simulink model "Koudruped_simcape"  (R2025b)
settings: Solver=VariableStepAuto  StartTime=0.0  StopTime=30  RelTol=1e-2
undefined symbols (not defined in the file or in its folder): fractalcoef, smiData, X, Y, Z
libraries: sm_lib x589, nesl_utility x93, slpidlib x5, mspsensorlib x4, simulink_extras x4, mspfiltlib x3, simulink x2
(part 3 of 16)

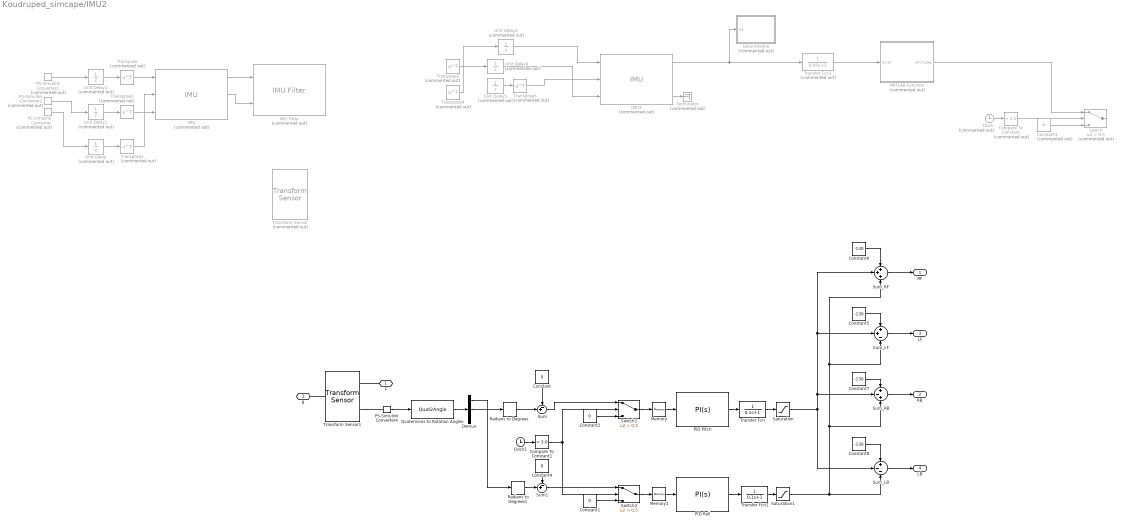
== system Koudruped_simcape/IMU2 ==
  Clock : Clock  Commented=on
  Clock1 : Clock
  Compare To Constant : simulink/Logic and Bit Operations/Compare To Constant  Commented=on  relop=>  const=3.0  OutDataTypeStr=boolean
  Compare To Constant1 : simulink/Logic and Bit Operations/Compare To Constant  relop=>  const=3.0  OutDataTypeStr=boolean
  Constant{,1..2,4} (4 alike) : Constant  Value=0
  Constant3 : Constant  Commented=on  Value=0
  Constant{5..8} (4 alike) : Constant  Value=-130
  Demux : Demux  Outputs=3
  Görüntüleme : Subsystem  Commented=on
  IMU : mspsensorlib/IMU  Commented=on  DispRefFrame=NED  TemperaturePort=off  Temperature=25  MagneticFieldPort=off  MagneticFieldNED=[ 27.5550, -2.4169, -16.0849 ]  MagneticFieldENU=[ -2.4169, 27.5550, 16.0849 ]  SeedDouble=67  SimulateUsing=Interpreted execution  AccelParamsMeasurementRange=156.96  AccelParamsResolution=0  AccelParamsConstantBias=[ 0.588, 0.588, 0.588 ]  AccelParamsAxesMisalignment=[ 100, 0, 0; 0, 100, 0; 0, 0, 100 ]  AccelParamsNoiseDensity=[ 0.00294, 0.00294, 0.00294 ]  AccelParamsBiasInstability=[ 0, 0, 0 ]  AccelParamsBiasInstabilityNumerator=fractalcoef().Numerator  AccelParamsBiasInstabilityDenominator=fractalcoef().Denominator  AccelParamsRandomWalk=[ 0, 0, 0 ]  AccelParamsNoiseType=double-sided  AccelParamsTemperatureBias=[ 0, 0, 0 ]  AccelParamsTemperatureScaleFactor=[ 0, 0, 0 ]  GyroParamsMeasurementRange=34.9  GyroParamsResolution=0  GyroParamsConstantBias=[ 0.0872, 0.0872, 0.0872 ]  GyroParamsAxesMisalignment=[ 100, 0, 0; 0, 100, 0; 0, 0, 100 ]  GyroParamsAccelerationBias=[ 0, 0, 0 ]  GyroParamsNoiseDensity=[ 0.0001745, 0.0001745, 0.0001745 ]  GyroParamsBiasInstability=[ 0, 0, 0 ]  GyroParamsBiasInstabilityNumerator=fractalcoef().Numerator  GyroParamsBiasInstabilityDenominator=fractalcoef().Denominator  GyroParamsRandomWalk=[ 0, 0, 0 ]  GyroParamsNoiseType=double-sided  GyroParamsTemperatureBias=[ 0, 0, 0 ]  GyroParamsTemperatureScaleFactor=[ 0, 0, 0 ]  MagParamsMeasurementRange=Inf  MagParamsResolution=0  MagParamsConstantBias=[ 0, 0, 0 ]  MagParamsAxesMisalignment=[ 100, 0, 0; 0, 100, 0; 0, 0, 100 ]  MagParamsNoiseDensity=[ 0, 0, 0 ]  MagParamsBiasInstability=[ 0, 0, 0 ]  MagParamsBiasInstabilityNumerator=fractalcoef().Numerator  MagParamsBiasInstabilityDenominator=fractalcoef().Denominator  MagParamsRandomWalk=[ 0, 0, 0 ]  MagParamsNoiseType=double-sided  MagParamsTemperatureBias=[ 0, 0, 0 ]  MagParamsTemperatureScaleFactor=[ 0, 0, 0 ]
  IMU Filter : mspfiltlib/IMU Filter  Commented=on  DispRefFrame=ENU  OrientationFormat=Rotation matrix  DecimationFactor=1  InitialProcessNoise=imufilter.defaultProcessNoise  AccelerometerNoise=8.64e-6  GyroscopeNoise=3.04e-8  GyroscopeDriftNoise=3.04e-13  LinearAccelerationNoise=0.0096236100000000012  LinearAccelerationDecayFactor=0.5  SimulateUsing=Interpreted execution
  IMU3 : mspsensorlib/IMU  Commented=on  DispRefFrame=ENU  TemperaturePort=off  Temperature=25  MagneticFieldPort=off  MagneticFieldNED=[ 27.5550, -2.4169, -16.0849 ]  MagneticFieldENU=[ -2.4169, 27.5550, 16.0849 ]  SeedDouble=67  SimulateUsing=Interpreted execution  AccelParamsMeasurementRange=19.6133  AccelParamsResolution=5.9855e-4  AccelParamsConstantBias=[ 0.19, 0.19, 0.19 ]  AccelParamsAxesMisalignment=[ 100, 0, 0; 0, 100, 0; 0, 0, 100 ]  AccelParamsNoiseDensity=[0.00294, 0.00294, 0.00294]  AccelParamsBiasInstability=[0.0004, 0.0004, 0.0004]  AccelParamsBiasInstabilityNumerator=fractalcoef().Numerator  AccelParamsBiasInstabilityDenominator=fractalcoef().Denominator  AccelParamsRandomWalk=[ 0, 0, 0 ]  AccelParamsNoiseType=double-sided  AccelParamsTemperatureBias=[ 0, 0, 0 ]  AccelParamsTemperatureScaleFactor=[ 0, 0, 0 ]  GyroParamsMeasurementRange=4.3633  GyroParamsResolution=0.00109  GyroParamsConstantBias=[0.0545, 0.0545, 0.0545]  GyroParamsAxesMisalignment=[ 100, 0, 0; 0, 100, 0; 0, 0, 100 ]  GyroParamsAccelerationBias=[ 0, 0, 0 ]  GyroParamsNoiseDensity=[4.36e-4, 4.36e-4, 4.36e-4]  GyroParamsBiasInstability=[2.4e-5, 2.4e-5, 2.4e-5]  GyroParamsBiasInstabilityNumerator=fractalcoef().Numerator  GyroParamsBiasInstabilityDenominator=fractalcoef().Denominator  GyroParamsRandomWalk=[ 0, 0, 0 ]  GyroParamsNoiseType=double-sided  GyroParamsTemperatureBias=[ 0, 0, 0 ]  GyroParamsTemperatureScaleFactor=[ 0, 0, 0 ]  MagParamsMeasurementRange=Inf  MagParamsResolution=0  MagParamsConstantBias=[ 0, 0, 0 ]  MagParamsAxesMisalignment=[ 100, 0, 0; 0, 100, 0; 0, 0, 100 ]  MagParamsNoiseDensity=[ 0, 0, 0 ]  MagParamsBiasInstability=[ 0, 0, 0 ]  MagParamsBiasInstabilityNumerator=fractalcoef().Numerator  MagParamsBiasInstabilityDenominator=fractalcoef().Denominator  MagParamsRandomWalk=[ 0, 0, 0 ]  MagParamsNoiseType=double-sided  MagParamsTemperatureBias=[ 0, 0, 0 ]  MagParamsTemperatureScaleFactor=[ 0, 0, 0 ]
  MATLAB Function : MATLAB Function  Commented=on  TreatAsAtomicUnit=on
  Memory : Memory
  Memory1 : Memory
  PID Pitch : slpidlib/PID Controller  Controller=PI  Form=Parallel  TimeDomain=Continuous-time  UseExternalTs=off  SampleTime=-1  IntegratorMethod=Forward Euler  FilterMethod=Forward Euler  ControllerParametersSource=internal  P=2  I=0.4  UseKiTs=off  D=0.05  UseExternalDerivativeSource=off  N=100  UseFilter=on  TunerSelectOption=Transfer Function Based (PID Tuner App)  InitialConditionSource=internal  InitialConditionForIntegrator=0  InitialConditionForFilter=0  DifferentiatorICPrevScaledInput=0  ExternalReset=none  TrackingMode=off  Kt=1  LimitOutput=on  SatLimitsSource=internal  UpperSaturationLimit=40  LowerSaturationLimit=-40  LinearizeAsGain=on  AntiWindupMode=back-calculation  Kb=1  LimitIntegrator=off  UpperIntegratorSaturationLimit=inf  LowerIntegratorSaturationLimit=-inf  POutMin=[]  POutMax=[]  IOutMin=[]  IOutMax=[]  DOutMin=[]  DOutMax=[]  NOutMin=[]  NOutMax=[]  SumOutMin=[]  SumOutMax=[]  SaturationOutMin=[]  SaturationOutMax=[]  PParamMin=[]  PParamMax=[]  IParamMin=[]  IParamMax=[]  DParamMin=[]  DParamMax=[]  NParamMin=[]  NParamMax=[]  KbParamMin=[]  KbParamMax=[]  KtParamMin=[]  KtParamMax=[]  KbOutMin=[]  KbOutMax=[]  KtOutMin=[]  KtOutMax=[]  IntegratorOutMin=[]  IntegratorOutMax=[]  FilterOutMin=[]  FilterOutMax=[]  SumI1OutMin=[]  SumI1OutMax=[]  SumI2OutMin=[]  SumI2OutMax=[]  SumI3OutMin=[]  SumI3OutMax=[]  SumI4OutMin=[]  SumI4OutMax=[]  SumDOutMin=[]  SumDOutMax=[]  DifferentiatorOutMin=[]  DifferentiatorOutMax=[]  FilterDiffOutCoefMin=[]  FilterDiffOutCoefMax=[]  ReciprocalOutMin=[]  ReciprocalOutMax=[]  SumDenOutMin=[]  SumDenOutMax=[]  SumNumOutMin=[]  SumNumOutMax=[]  DivideOutMin=[]  DivideOutMax=[]  UdiffTsProdOutMin=[]  UdiffTsProdOutMax=[]  NTsProdOutMin=[]  NTsProdOutMax=[]  UintegralTsProdOutMin=[]  UintegralTsProdOutMax=[]  UngainTsProdOutMin=[]  UngainTsProdOutMax=[]  ClampingZeroOutDataTypeStr=Inherit: Inherit via back propagation  ClampingZeroOutMin=[]  ClampingZeroOutMax=[]  FilterDenConstantOutDataTypeStr=Inherit: Inherit via back propagation  FilterDenConstantOutMin=[]  FilterDenConstantOutMax=[]  PCopyOutDataTypeStr=Inherit: Inherit via back propagation  PCopyOutMin=[]  PCopyOutMax=[]  NCopyOutDataTypeStr=Inherit: Inherit via back propagation  NCopyOutMin=[]  NCopyOutMax=[]  IntegratorContinuousStateAttributes=''  IntegratorStateMustResolveToSignalObject=off  IntegratorRTWStateStorageClass=Auto  FilterContinuousStateAttributes=''  FilterStateMustResolveToSignalObject=off  FilterRTWStateStorageClass=Auto  ParallelPVariant=InternalParameters  IdealPVariant=Disabled  IVariant=InternalParameters  DVariant=Disabled  IntegratorVariant=Continuous  SatVariant=Enabled  AWVariant=BackCalculation  PCopyVariant=Disabled  TRVariant=Disabled  FdbkBlocksVariant=Forward  IdealPFdbkVariant=Disabled  SatFdbkVariant=Disabled  DerivativeFilterVariant=Disabled  NVariant=Disabled  NCopyVariant=Disabled_SignalSpec  FilterICVariant=Disabled  IntegratorICVariant=InternalICs  ExternalResetVariant=Disabled  TRSumVariant=Passthrough  SumFdbkVariant=Disabled  SumVariant=Sum_PI  TsampFilterVariant=InternalTs  TsampNgainVariant=Passthrough  TsampIntegralVariant=Disabled_SignalSpec  ExternalSaturationOutDataTypeStr=Inherit: Same as second input  DerivativeSourceVariant=Disabled  PreIntVariant=InternalPreInt
  PID Roll : slpidlib/PID Controller  Controller=PI  Form=Parallel  TimeDomain=Continuous-time  UseExternalTs=off  SampleTime=-1  IntegratorMethod=Forward Euler  FilterMethod=Forward Euler  ControllerParametersSource=internal  P=2  I=0.4  UseKiTs=off  D=0.05  UseExternalDerivativeSource=off  N=100  UseFilter=on  TunerSelectOption=Transfer Function Based (PID Tuner App)  InitialConditionSource=internal  InitialConditionForIntegrator=0  InitialConditionForFilter=0  DifferentiatorICPrevScaledInput=0  ExternalReset=none  TrackingMode=off  Kt=1  LimitOutput=on  SatLimitsSource=internal  UpperSaturationLimit=40  LowerSaturationLimit=-40  LinearizeAsGain=on  AntiWindupMode=back-calculation  Kb=1  LimitIntegrator=off  UpperIntegratorSaturationLimit=inf  LowerIntegratorSaturationLimit=-inf  POutMin=[]  POutMax=[]  IOutMin=[]  IOutMax=[]  DOutMin=[]  DOutMax=[]  NOutMin=[]  NOutMax=[]  SumOutMin=[]  SumOutMax=[]  SaturationOutMin=[]  SaturationOutMax=[]  PParamMin=[]  PParamMax=[]  IParamMin=[]  IParamMax=[]  DParamMin=[]  DParamMax=[]  NParamMin=[]  NParamMax=[]  KbParamMin=[]  KbParamMax=[]  KtParamMin=[]  KtParamMax=[]  KbOutMin=[]  KbOutMax=[]  KtOutMin=[]  KtOutMax=[]  IntegratorOutMin=[]  IntegratorOutMax=[]  FilterOutMin=[]  FilterOutMax=[]  SumI1OutMin=[]  SumI1OutMax=[]  SumI2OutMin=[]  SumI2OutMax=[]  SumI3OutMin=[]  SumI3OutMax=[]  SumI4OutMin=[]  SumI4OutMax=[]  SumDOutMin=[]  SumDOutMax=[]  DifferentiatorOutMin=[]  DifferentiatorOutMax=[]  FilterDiffOutCoefMin=[]  FilterDiffOutCoefMax=[]  ReciprocalOutMin=[]  ReciprocalOutMax=[]  SumDenOutMin=[]  SumDenOutMax=[]  SumNumOutMin=[]  SumNumOutMax=[]  DivideOutMin=[]  DivideOutMax=[]  UdiffTsProdOutMin=[]  UdiffTsProdOutMax=[]  NTsProdOutMin=[]  NTsProdOutMax=[]  UintegralTsProdOutMin=[]  UintegralTsProdOutMax=[]  UngainTsProdOutMin=[]  UngainTsProdOutMax=[]  ClampingZeroOutDataTypeStr=Inherit: Inherit via back propagation  ClampingZeroOutMin=[]  ClampingZeroOutMax=[]  FilterDenConstantOutDataTypeStr=Inherit: Inherit via back propagation  FilterDenConstantOutMin=[]  FilterDenConstantOutMax=[]  PCopyOutDataTypeStr=Inherit: Inherit via back propagation  PCopyOutMin=[]  PCopyOutMax=[]  NCopyOutDataTypeStr=Inherit: Inherit via back propagation  NCopyOutMin=[]  NCopyOutMax=[]  IntegratorContinuousStateAttributes=''  IntegratorStateMustResolveToSignalObject=off  IntegratorRTWStateStorageClass=Auto  FilterContinuousStateAttributes=''  FilterStateMustResolveToSignalObject=off  FilterRTWStateStorageClass=Auto  ParallelPVariant=InternalParameters  IdealPVariant=Disabled  IVariant=InternalParameters  DVariant=Disabled  IntegratorVariant=Continuous  SatVariant=Enabled  AWVariant=BackCalculation  PCopyVariant=Disabled  TRVariant=Disabled  FdbkBlocksVariant=Forward  IdealPFdbkVariant=Disabled  SatFdbkVariant=Disabled  DerivativeFilterVariant=Disabled  NVariant=Disabled  NCopyVariant=Disabled_SignalSpec  FilterICVariant=Disabled  IntegratorICVariant=InternalICs  ExternalResetVariant=Disabled  TRSumVariant=Passthrough  SumFdbkVariant=Disabled  SumVariant=Sum_PI  TsampFilterVariant=InternalTs  TsampNgainVariant=Passthrough  TsampIntegralVariant=Disabled_SignalSpec  ExternalSaturationOutDataTypeStr=Inherit: Same as second input  DerivativeSourceVariant=Disabled  PreIntVariant=InternalPreInt
  PS-Simulink Converter : nesl_utility/PS-Simulink Converter  Commented=on  PhysicalDomain=network_engine_domain  SubClassName=ps_output  LeftPortType=input  RightPortType=output  PseudoPeriodic=off  Frequencies=[]  VectorFormat=inherit  Unit=inherit  AffineConversion=off
  PS-Simulink Converter1 : nesl_utility/PS-Simulink Converter  Commented=on  PhysicalDomain=network_engine_domain  SubClassName=ps_output  LeftPortType=input  RightPortType=output  PseudoPeriodic=off  Frequencies=[]  VectorFormat=inherit  Unit=inherit  AffineConversion=off
  PS-Simulink Converter2 : nesl_utility/PS-Simulink Converter  Commented=on  PhysicalDomain=network_engine_domain  SubClassName=ps_output  LeftPortType=input  RightPortType=output  PseudoPeriodic=off  Frequencies=[]  VectorFormat=inherit  Unit=inherit  AffineConversion=off
  PS-Simulink Converter4 : nesl_utility/PS-Simulink Converter  PhysicalDomain=network_engine_domain  SubClassName=ps_output  LeftPortType=input  RightPortType=output  PseudoPeriodic=off  Frequencies=[]  VectorFormat=inherit  Unit=inherit  AffineConversion=off
  Quaternions to Rotation Angles : Quat2Angle
      settings: AttributesFormatString=Rotation Order: %<rotationOrder>
  Radians to Degrees : simulink_extras/Transformations/Radians to Degrees
  Radians to Degrees1 : simulink_extras/Transformations/Radians to Degrees
  Saturation : Saturate  UpperLimit=+40  LowerLimit=-40
  Saturation1 : Saturate  UpperLimit=+40  LowerLimit=-40
  Sum : Sum  Inputs=-+|
  Sum1 : Sum  Inputs=-+|
  Sum_LB : Sum  Inputs=+--
  Sum_LF : Sum  Inputs=++-
  Sum_RB : Sum  Inputs=+-+
  Sum_RF : Sum  Inputs=+++
  Switch : Switch  Commented=on  Criteria=u2 > Threshold  Threshold=0.5  SaturateOnIntegerOverflow=off  InputSameDT=off
  Switch1 : Switch  Criteria=u2 > Threshold  Threshold=0.5  SaturateOnIntegerOverflow=off  InputSameDT=off
  Switch2 : Switch  Criteria=u2 > Threshold  Threshold=0.5  SaturateOnIntegerOverflow=off  InputSameDT=off
  Terminator : Terminator  Commented=on
  Transfer Fcn : TransferFcn  Denominator=[0.1 1]
  Transfer Fcn1 : TransferFcn  Commented=on  Denominator=[0.05 1]
  Transfer Fcn2 : TransferFcn  Denominator=[0.1 1]
  Transform Sensor : sm_lib/Frames and Transforms/Transform Sensor  Commented=on  MeasurementFrame=World  RotationSequence=ZYX  SenseAngle=off  SenseAxis=off  SenseQ=on  SenseR=off  SenseRotationSequence=off  SenseOmegaX=off  SenseOmegaY=off  SenseOmegaZ=off  SenseOmega=on  SenseQDot=off  SenseRDot=off  SenseRotationSequenceDot=off  SenseAlphaX=off  SenseAlphaY=off  SenseAlphaZ=off  SenseAlpha=off  SenseQDDot=off  SenseRDDot=off  SenseX=off  SenseY=off  SenseZ=off  SenseXYZ=off  SenseRad=off  SenseAzim=off  SenseDist=off  SenseInc=off  SenseXDot=off  SenseYDot=off  SenseZDot=off  SenseXYZDot=off  SenseRadDot=off  SenseAzimDot=off  SenseDistDot=off  SenseIncDot=off  SenseXDDot=off  SenseYDDot=off  SenseZDDot=off  SenseXYZDDot=on  SenseRadDDot=off  SenseAzimDDot=off  SenseDistDDot=off  SenseIncDDot=off
  Transform Sensor1 : sm_lib/Frames and Transforms/Transform Sensor  MeasurementFrame=World  RotationSequence=ZYX  SenseAngle=off  SenseAxis=off  SenseQ=on  SenseR=off  SenseRotationSequence=off  SenseOmegaX=off  SenseOmegaY=off  SenseOmegaZ=off  SenseOmega=off  SenseQDot=off  SenseRDot=off  SenseRotationSequenceDot=off  SenseAlphaX=off  SenseAlphaY=off  SenseAlphaZ=off  SenseAlpha=off  SenseQDDot=off  SenseRDDot=off  SenseX=off  SenseY=off  SenseZ=off  SenseXYZ=off  SenseRad=off  SenseAzim=off  SenseDist=off  SenseInc=off  SenseXDot=off  SenseYDot=off  SenseZDot=off  SenseXYZDot=off  SenseRadDot=off  SenseAzimDot=off  SenseDistDot=off  SenseIncDot=off  SenseXDDot=off  SenseYDDot=off  SenseZDDot=off  SenseXYZDDot=off  SenseRadDDot=off  SenseAzimDDot=off  SenseDistDDot=off  SenseIncDDot=off
  Transpose{,1..5} (6 alike) : Math  Commented=on  Operator=transpose
  Unit Delay : UnitDelay  Commented=on  SampleTime=-1  HasFrameUpgradeWarning=on
  Unit Delay1 : UnitDelay  Commented=on  InitialCondition="[1 0 0 ;0 0 0  ; 0 0 0 ]"  SampleTime=-1  HasFrameUpgradeWarning=on
  Unit Delay2 : UnitDelay  Commented=on  InitialCondition=[0 ;0 ;-9.81 ]  SampleTime=-1  HasFrameUpgradeWarning=on
  Unit Delay3 : UnitDelay  Commented=on  SampleTime=0.001  HasFrameUpgradeWarning=on
  Unit Delay4 : UnitDelay  Commented=on  SampleTime=0.001  HasFrameUpgradeWarning=on
  Unit Delay5 : UnitDelay  Commented=on  SampleTime=0.001  HasFrameUpgradeWarning=on
  F : PMIOPort  Side=Left
  B : PMIOPort  Port=2  Side=Left
  RF : Outport
  RB : Outport  Port=2
  LF : Outport  Port=3
  LB : Outport  Port=4
  wires:
  Constant/1 -> Sum/1
  PID Pitch/1 -> Transfer Fcn/1
  Demux/2 -> Radians to Degrees/1
  Quaternions to Rotation Angles/1 -> Demux/1
  Transpose2/1 -> IMU/3
  Unit Delay2/1 -> Transpose/1
  PS-Simulink Converter1/1 -> Unit Delay2/1
  PS-Simulink Converter2/1 -> Unit Delay1/1
  Unit Delay1/1 -> Transpose2/1
  PS-Simulink Converter/1 -> Unit Delay/1
  IMU/2 -> IMU Filter/2
  Unit Delay/1 -> Transpose1/1
  IMU/1 -> IMU Filter/1
  Transpose/1 -> IMU/1
  Transpose1/1 -> IMU/2
  Memory/1 -> PID Pitch/1
  Transfer Fcn/1 -> Saturation/1
  Transpose4/1 -> Unit Delay3/1
  Transpose3/1 -> IMU3/2
  Transpose5/1 -> Unit Delay4/1
  Unit Delay3/1 -> IMU3/1
  Unit Delay4/1 -> IMU3/3
  Unit Delay5/1 -> Transpose3/1
  IMU3/1 -> Transfer Fcn1/1, Görüntüleme/1(In1)
  IMU3/3 -> Terminator/1
  Compare To Constant/1 -> Switch/2
  Constant3/1 -> Switch/3
  Clock/1 -> Compare To Constant/1
  Transfer Fcn1/1 -> MATLAB Function/1(accel)
  MATLAB Function/1(pitch_deg) -> Switch/1
  Radians to Degrees/1 -> Sum/2
  PS-Simulink Converter4/1 -> Quaternions to Rotation Angles/1
  Radians to Degrees1/1 -> Sum1/2
  PID Roll/1 -> Transfer Fcn2/1
  Memory1/1 -> PID Roll/1
  Constant4/1 -> Sum1/1
  Transfer Fcn2/1 -> Saturation1/1
  Sum_RF/1 -> RF/1
  Sum_LF/1 -> LF/1
  Sum_RB/1 -> RB/1
  Sum_LB/1 -> LB/1
  Constant5/1 -> Sum_LF/1
  Constant6/1 -> Sum_RF/1
  Constant7/1 -> Sum_RB/1
  Constant8/1 -> Sum_LB/1
  Saturation/1 -> Sum_LB/2, Sum_LF/2, Sum_RF/2, Sum_RB/2
  Saturation1/1 -> Sum_RB/3, Sum_LF/3, Sum_RF/3, Sum_LB/3
  Clock1/1 -> Compare To Constant1/1
  Constant2/1 -> Switch1/3
  Switch2/1 -> Memory1/1
  Constant1/1 -> Switch2/3
  Compare To Constant1/1 -> Switch1/2, Switch2/2
  Switch1/1 -> Memory/1
  Sum/1 -> Switch1/1
  Sum1/1 -> Switch2/1
  Demux/1 -> Radians to Degrees1/1
  connections:
  Transform Sensor1/LConn1 -- B/RConn1
  Transform Sensor1/RConn2 -- PS-Simulink Converter4/LConn1
  F/RConn1 -- Transform Sensor1/RConn1

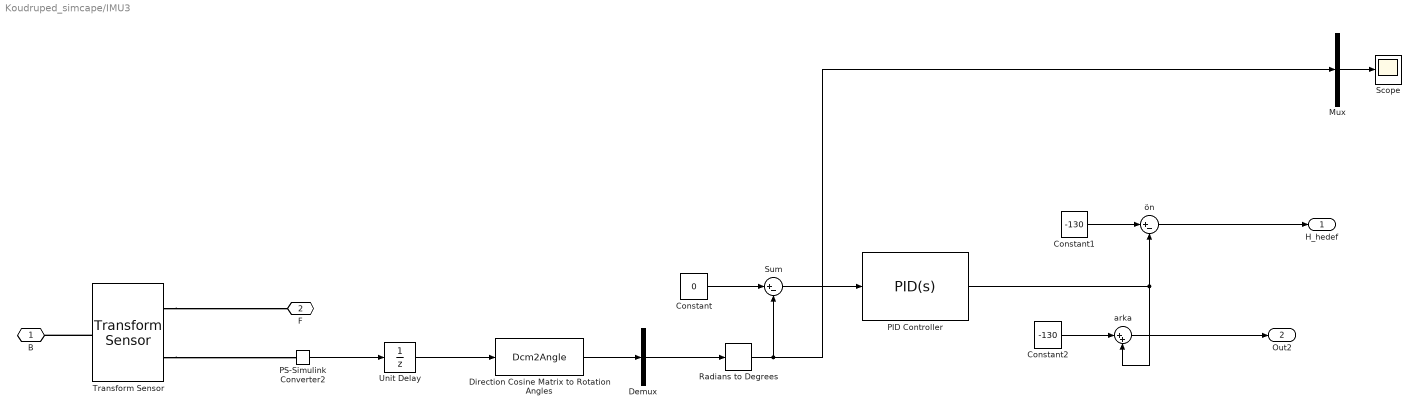
== system Koudruped_simcape/IMU3 ==
  Constant : Constant  Value=0
  Constant1 : Constant  Value=-130
  Constant2 : Constant  Value=-130
  Demux : Demux  Outputs=3
  Direction Cosine Matrix to Rotation Angles : Dcm2Angle
      settings: AttributesFormatString=Rotation Order: %<rotationOrder>
  Mux : Mux  Inputs=3
  PID Controller : slpidlib/PID Controller  Controller=PID  Form=Parallel  TimeDomain=Continuous-time  UseExternalTs=off  SampleTime=-1  IntegratorMethod=Forward Euler  FilterMethod=Forward Euler  ControllerParametersSource=internal  P=1  I=0.05  UseKiTs=off  D=0  UseExternalDerivativeSource=off  N=100  UseFilter=on  TunerSelectOption=Transfer Function Based (PID Tuner App)  InitialConditionSource=internal  InitialConditionForIntegrator=0  InitialConditionForFilter=0  DifferentiatorICPrevScaledInput=0  ExternalReset=none  TrackingMode=off  Kt=1  LimitOutput=off  SatLimitsSource=internal  UpperSaturationLimit=inf  LowerSaturationLimit=-inf  LinearizeAsGain=on  AntiWindupMode=none  Kb=1  LimitIntegrator=off  UpperIntegratorSaturationLimit=inf  LowerIntegratorSaturationLimit=-inf  POutMin=[]  POutMax=[]  IOutMin=[]  IOutMax=[]  DOutMin=[]  DOutMax=[]  NOutMin=[]  NOutMax=[]  SumOutMin=[]  SumOutMax=[]  SaturationOutMin=[]  SaturationOutMax=[]  PParamMin=[]  PParamMax=[]  IParamMin=[]  IParamMax=[]  DParamMin=[]  DParamMax=[]  NParamMin=[]  NParamMax=[]  KbParamMin=[]  KbParamMax=[]  KtParamMin=[]  KtParamMax=[]  KbOutMin=[]  KbOutMax=[]  KtOutMin=[]  KtOutMax=[]  IntegratorOutMin=[]  IntegratorOutMax=[]  FilterOutMin=[]  FilterOutMax=[]  SumI1OutMin=[]  SumI1OutMax=[]  SumI2OutMin=[]  SumI2OutMax=[]  SumI3OutMin=[]  SumI3OutMax=[]  SumI4OutMin=[]  SumI4OutMax=[]  SumDOutMin=[]  SumDOutMax=[]  DifferentiatorOutMin=[]  DifferentiatorOutMax=[]  FilterDiffOutCoefMin=[]  FilterDiffOutCoefMax=[]  ReciprocalOutMin=[]  ReciprocalOutMax=[]  SumDenOutMin=[]  SumDenOutMax=[]  SumNumOutMin=[]  SumNumOutMax=[]  DivideOutMin=[]  DivideOutMax=[]  UdiffTsProdOutMin=[]  UdiffTsProdOutMax=[]  NTsProdOutMin=[]  NTsProdOutMax=[]  UintegralTsProdOutMin=[]  UintegralTsProdOutMax=[]  UngainTsProdOutMin=[]  UngainTsProdOutMax=[]  ClampingZeroOutDataTypeStr=Inherit: Inherit via back propagation  ClampingZeroOutMin=[]  ClampingZeroOutMax=[]  FilterDenConstantOutDataTypeStr=Inherit: Inherit via back propagation  FilterDenConstantOutMin=[]  FilterDenConstantOutMax=[]  PCopyOutDataTypeStr=Inherit: Inherit via back propagation  PCopyOutMin=[]  PCopyOutMax=[]  NCopyOutDataTypeStr=Inherit: Inherit via back propagation  NCopyOutMin=[]  NCopyOutMax=[]  IntegratorContinuousStateAttributes=''  IntegratorStateMustResolveToSignalObject=off  IntegratorRTWStateStorageClass=Auto  FilterContinuousStateAttributes=''  FilterStateMustResolveToSignalObject=off  FilterRTWStateStorageClass=Auto  ParallelPVariant=InternalParameters  IdealPVariant=Disabled  IVariant=InternalParameters  DVariant=InternalParameters  IntegratorVariant=Continuous  SatVariant=Disabled  AWVariant=Passthrough  PCopyVariant=Disabled  TRVariant=Disabled  FdbkBlocksVariant=Forward  IdealPFdbkVariant=Disabled  SatFdbkVariant=Disabled  DerivativeFilterVariant=ContFilter  NVariant=InternalParameters  NCopyVariant=Disabled  FilterICVariant=InternalICsFilter  IntegratorICVariant=InternalICs  ExternalResetVariant=Disabled  TRSumVariant=Passthrough  SumFdbkVariant=Disabled  SumVariant=Sum_PID  TsampFilterVariant=InternalTs  TsampNgainVariant=Passthrough  TsampIntegralVariant=Disabled_SignalSpec  ExternalSaturationOutDataTypeStr=Inherit: Same as second input  DerivativeSourceVariant=ErrorSignal  PreIntVariant=InternalPreInt
  PS-Simulink Converter2 : nesl_utility/PS-Simulink Converter  PhysicalDomain=network_engine_domain  SubClassName=ps_output  LeftPortType=input  RightPortType=output  PseudoPeriodic=off  Frequencies=[]  VectorFormat=inherit  Unit=inherit  AffineConversion=off
  Radians to Degrees : simulink_extras/Transformations/Radians to Degrees
  Scope : Scope
      settings: ActiveDisplayYMinimum=-51.725776270156686  ActiveDisplayYMaximum=42.428044280294451  DataLoggingVariableName=ScopeData2
  Sum : Sum  Inputs=|+-
  Transform Sensor : sm_lib/Frames and Transforms/Transform Sensor  MeasurementFrame=World  RotationSequence=XYX  SenseAngle=off  SenseAxis=off  SenseQ=off  SenseR=on  SenseRotationSequence=off  SenseOmegaX=off  SenseOmegaY=off  SenseOmegaZ=off  SenseOmega=off  SenseQDot=off  SenseRDot=off  SenseRotationSequenceDot=off  SenseAlphaX=off  SenseAlphaY=off  SenseAlphaZ=off  SenseAlpha=off  SenseQDDot=off  SenseRDDot=off  SenseX=off  SenseY=off  SenseZ=off  SenseXYZ=off  SenseRad=off  SenseAzim=off  SenseDist=off  SenseInc=off  SenseXDot=off  SenseYDot=off  SenseZDot=off  SenseXYZDot=off  SenseRadDot=off  SenseAzimDot=off  SenseDistDot=off  SenseIncDot=off  SenseXDDot=off  SenseYDDot=off  SenseZDDot=off  SenseXYZDDot=off  SenseRadDDot=off  SenseAzimDDot=off  SenseDistDDot=off  SenseIncDDot=off
  Unit Delay : UnitDelay  SampleTime=-1  HasFrameUpgradeWarning=on
  arka : Sum  Inputs=|++
  ön : Sum  Inputs=|+-
  B : PMIOPort  Side=Left
  F : PMIOPort  Port=2  Side=Left
  H_hedef : Outport
  Out2 : Outport  Port=2
  wires:
  ön/1 -> H_hedef/1
  Constant/1 -> Sum/1
  Constant2/1 -> arka/1
  Constant1/1 -> ön/1
  PID Controller/1 -> ön/2, arka/2
  Sum/1 -> PID Controller/1
  Demux/2 -> Radians to Degrees/1
  Direction Cosine Matrix to Rotation Angles/1 -> Demux/1
  Radians to Degrees/1 -> Mux/2, Sum/2
  PS-Simulink Converter2/1 -> Unit Delay/1
  Unit Delay/1 -> Direction Cosine Matrix to Rotation Angles/1
  arka/1 -> Out2/1
  Mux/1 -> Scope/1
  connections:
  Transform Sensor/RConn2 -- PS-Simulink Converter2/LConn1
  Transform Sensor/LConn1 -- B/RConn1
  Transform Sensor/RConn1 -- F/RConn1

== system Koudruped_simcape/Left Back Step ==
  H_hedef : Inport
  Clock1 : Clock
  Constant : Constant  Value=0
  Demux1 : Demux  Outputs=3
  Gain : Gain  Gain=-1
  MATLAB Function1 : MATLAB Function  TreatAsAtomicUnit=on
  MATLAB Function2 : MATLAB Function  TreatAsAtomicUnit=on
  Simulink-PS Converter1 : nesl_utility/Simulink-PS Converter  PhysicalDomain=network_engine_domain  SubClassName=ps_input  LeftPortType=input  RightPortType=output  PseudoPeriodic=off  Frequencies=[]  NoiseDistribution=none  NoiseParameters=[]  Unit=deg  AffineConversion=off  FilteringAndDerivatives=filter  SimscapeFilterOrder=2  InputFilterTimeConstant=0.001  UdotUserProvided=0
  Simulink-PS Converter2 : nesl_utility/Simulink-PS Converter  PhysicalDomain=network_engine_domain  SubClassName=ps_input  LeftPortType=input  RightPortType=output  PseudoPeriodic=off  Frequencies=[]  NoiseDistribution=none  NoiseParameters=[]  Unit=deg  AffineConversion=off  FilteringAndDerivatives=filter  SimscapeFilterOrder=2  InputFilterTimeConstant=0.001  UdotUserProvided=0
  Simulink-PS Converter3 : nesl_utility/Simulink-PS Converter  PhysicalDomain=network_engine_domain  SubClassName=ps_input  LeftPortType=input  RightPortType=output  PseudoPeriodic=off  Frequencies=[]  NoiseDistribution=none  NoiseParameters=[]  Unit=deg  AffineConversion=off  FilteringAndDerivatives=filter  SimscapeFilterOrder=2  InputFilterTimeConstant=0.001  UdotUserProvided=0
  Mafsal 1 : PMIOPort  Side=Right
  Mafsal 2 : PMIOPort  Port=2  Side=Right
  Mafsal 3 : PMIOPort  Port=3  Side=Right
  wires:
  Clock1/1 -> MATLAB Function1/1(t)
  Constant/1 -> MATLAB Function1/2(phase_offset)
  MATLAB Function1/1(pos) -> MATLAB Function2/1(pos)
  Demux1/2 -> Simulink-PS Converter1/1
  Demux1/3 -> Simulink-PS Converter2/1
  Demux1/1 -> Gain/1
  MATLAB Function2/1(angles) -> Demux1/1
  H_hedef/1 -> MATLAB Function1/3(H_hedef)
  Gain/1 -> Simulink-PS Converter3/1
  connections:
  Mafsal 1/RConn1 -- Simulink-PS Converter3/RConn1
  Simulink-PS Converter1/RConn1 -- Mafsal 2/RConn1
  Simulink-PS Converter2/RConn1 -- Mafsal 3/RConn1

== system Koudruped_simcape/Left Back Step1 ==
  H_hedef : Inport
  Clock1 : Clock
  Constant : Constant  Value=0
  Demux1 : Demux  Outputs=3
  Gain : Gain  Gain=-1
  MATLAB Function1 : MATLAB Function  TreatAsAtomicUnit=on
  MATLAB Function2 : MATLAB Function  TreatAsAtomicUnit=on
  Simulink-PS Converter1 : nesl_utility/Simulink-PS Converter  PhysicalDomain=network_engine_domain  SubClassName=ps_input  LeftPortType=input  RightPortType=output  PseudoPeriodic=off  Frequencies=[]  NoiseDistribution=none  NoiseParameters=[]  Unit=deg  AffineConversion=off  FilteringAndDerivatives=filter  SimscapeFilterOrder=2  InputFilterTimeConstant=0.001  UdotUserProvided=0
  Simulink-PS Converter2 : nesl_utility/Simulink-PS Converter  PhysicalDomain=network_engine_domain  SubClassName=ps_input  LeftPortType=input  RightPortType=output  PseudoPeriodic=off  Frequencies=[]  NoiseDistribution=none  NoiseParameters=[]  Unit=deg  AffineConversion=off  FilteringAndDerivatives=filter  SimscapeFilterOrder=2  InputFilterTimeConstant=0.001  UdotUserProvided=0
  Simulink-PS Converter3 : nesl_utility/Simulink-PS Converter  PhysicalDomain=network_engine_domain  SubClassName=ps_input  LeftPortType=input  RightPortType=output  PseudoPeriodic=off  Frequencies=[]  NoiseDistribution=none  NoiseParameters=[]  Unit=deg  AffineConversion=off  FilteringAndDerivatives=filter  SimscapeFilterOrder=2  InputFilterTimeConstant=0.001  UdotUserProvided=0
  Mafsal 1 : PMIOPort  Side=Right
  Mafsal 2 : PMIOPort  Port=2  Side=Right
  Mafsal 3 : PMIOPort  Port=3  Side=Right
  wires:
  Clock1/1 -> MATLAB Function1/1(t)
  Constant/1 -> MATLAB Function1/2(phase_offset)
  MATLAB Function1/1(pos) -> MATLAB Function2/1(pos)
  Demux1/2 -> Simulink-PS Converter1/1
  Demux1/1 -> Gain/1
  MATLAB Function2/1(angles) -> Demux1/1
  H_hedef/1 -> MATLAB Function1/3(H_hedef)
  Gain/1 -> Simulink-PS Converter3/1
  Demux1/3 -> Simulink-PS Converter2/1
  connections:
  Mafsal 1/RConn1 -- Simulink-PS Converter3/RConn1
  Simulink-PS Converter1/RConn1 -- Mafsal 2/RConn1
  Simulink-PS Converter2/RConn1 -- Mafsal 3/RConn1

== system Koudruped_simcape/Left Back Step2 ==
  H_hedef : Inport
  Clock1 : Clock
  Constant : Constant  Value=0
  Demux1 : Demux  Outputs=3
  Display : Display
  Gain : Gain  Gain=-1
  Left Back : Scope
      settings: ActiveDisplayYMinimum=-1  ActiveDisplayYMaximum=1  DataLoggingVariableName=ScopeData4
  Left Back1 : Scope
      settings: ActiveDisplayYMinimum=-1  ActiveDisplayYMaximum=1  DataLoggingVariableName=ScopeData5
  MATLAB Function1 : MATLAB Function  TreatAsAtomicUnit=on
  MATLAB Function2 : MATLAB Function  TreatAsAtomicUnit=on
  Simulink-PS Converter1 : nesl_utility/Simulink-PS Converter  PhysicalDomain=network_engine_domain  SubClassName=ps_input  LeftPortType=input  RightPortType=output  PseudoPeriodic=off  Frequencies=[]  NoiseDistribution=none  NoiseParameters=[]  Unit=deg  AffineConversion=off  FilteringAndDerivatives=filter  SimscapeFilterOrder=2  InputFilterTimeConstant=0.001  UdotUserProvided=0
  Simulink-PS Converter2 : nesl_utility/Simulink-PS Converter  PhysicalDomain=network_engine_domain  SubClassName=ps_input  LeftPortType=input  RightPortType=output  PseudoPeriodic=off  Frequencies=[]  NoiseDistribution=none  NoiseParameters=[]  Unit=deg  AffineConversion=off  FilteringAndDerivatives=filter  SimscapeFilterOrder=2  InputFilterTimeConstant=0.001  UdotUserProvided=0
  Simulink-PS Converter3 : nesl_utility/Simulink-PS Converter  PhysicalDomain=network_engine_domain  SubClassName=ps_input  LeftPortType=input  RightPortType=output  PseudoPeriodic=off  Frequencies=[]  NoiseDistribution=none  NoiseParameters=[]  Unit=deg  AffineConversion=off  FilteringAndDerivatives=filter  SimscapeFilterOrder=2  InputFilterTimeConstant=0.001  UdotUserProvided=0
  Mafsal 1 : PMIOPort  Side=Right
  Mafsal 2 : PMIOPort  Port=2  Side=Right
  Mafsal 3 : PMIOPort  Port=3  Side=Right
  wires:
  Clock1/1 -> MATLAB Function1/1(t)
  Constant/1 -> MATLAB Function1/2(phase_offset)
  MATLAB Function1/1(pos) -> MATLAB Function2/1(pos)
  Demux1/2 -> Simulink-PS Converter1/1
  Demux1/1 -> Gain/1
  MATLAB Function2/1(angles) -> Demux1/1
  H_hedef/1 -> Display/1, Left Back/1, MATLAB Function1/3(H_hedef)
  Gain/1 -> Simulink-PS Converter3/1
  Demux1/3 -> Left Back1/1, Simulink-PS Converter2/1
  connections:
  Mafsal 1/RConn1 -- Simulink-PS Converter3/RConn1
  Simulink-PS Converter1/RConn1 -- Mafsal 2/RConn1
  Simulink-PS Converter2/RConn1 -- Mafsal 3/RConn1

== system Koudruped_simcape/Left Back Step3 ==
  H_hedef : Inport
  Clock1 : Clock
  Constant : Constant  Value=0
  Demux1 : Demux  Outputs=3
  Gain : Gain  Gain=-1
  MATLAB Function1 : MATLAB Function  TreatAsAtomicUnit=on
  MATLAB Function2 : MATLAB Function  TreatAsAtomicUnit=on
  Simulink-PS Converter1 : nesl_utility/Simulink-PS Converter  PhysicalDomain=network_engine_domain  SubClassName=ps_input  LeftPortType=input  RightPortType=output  PseudoPeriodic=off  Frequencies=[]  NoiseDistribution=none  NoiseParameters=[]  Unit=deg  AffineConversion=off  FilteringAndDerivatives=filter  SimscapeFilterOrder=2  InputFilterTimeConstant=0.001  UdotUserProvided=0
  Simulink-PS Converter2 : nesl_utility/Simulink-PS Converter  PhysicalDomain=network_engine_domain  SubClassName=ps_input  LeftPortType=input  RightPortType=output  PseudoPeriodic=off  Frequencies=[]  NoiseDistribution=none  NoiseParameters=[]  Unit=deg  AffineConversion=off  FilteringAndDerivatives=filter  SimscapeFilterOrder=2  InputFilterTimeConstant=0.001  UdotUserProvided=0
  Simulink-PS Converter3 : nesl_utility/Simulink-PS Converter  PhysicalDomain=network_engine_domain  SubClassName=ps_input  LeftPortType=input  RightPortType=output  PseudoPeriodic=off  Frequencies=[]  NoiseDistribution=none  NoiseParameters=[]  Unit=deg  AffineConversion=off  FilteringAndDerivatives=filter  SimscapeFilterOrder=2  InputFilterTimeConstant=0.001  UdotUserProvided=0
  Mafsal 1 : PMIOPort  Side=Right
  Mafsal 2 : PMIOPort  Port=2  Side=Right
  Mafsal 3 : PMIOPort  Port=3  Side=Right
  wires:
  Clock1/1 -> MATLAB Function1/1(t)
  Constant/1 -> MATLAB Function1/2(phase_offset)
  MATLAB Function1/1(pos) -> MATLAB Function2/1(pos)
  Demux1/2 -> Simulink-PS Converter1/1
  Demux1/1 -> Gain/1
  MATLAB Function2/1(angles) -> Demux1/1
  H_hedef/1 -> MATLAB Function1/3(H_hedef)
  Gain/1 -> Simulink-PS Converter3/1
  Demux1/3 -> Simulink-PS Converter2/1
  connections:
  Mafsal 1/RConn1 -- Simulink-PS Converter3/RConn1
  Simulink-PS Converter1/RConn1 -- Mafsal 2/RConn1
  Simulink-PS Converter2/RConn1 -- Mafsal 3/RConn1

== system Koudruped_simcape/Left Front Step ==
  H_hedef : Inport
  Clock1 : Clock
  Constant : Constant  Value=0.5
  Demux1 : Demux  Outputs=3
  Gain : Gain  Gain=-1
  MATLAB Function1 : MATLAB Function  TreatAsAtomicUnit=on
  MATLAB Function2 : MATLAB Function  TreatAsAtomicUnit=on
  Simulink-PS Converter1 : nesl_utility/Simulink-PS Converter  PhysicalDomain=network_engine_domain  SubClassName=ps_input  LeftPortType=input  RightPortType=output  PseudoPeriodic=off  Frequencies=[]  NoiseDistribution=none  NoiseParameters=[]  Unit=deg  AffineConversion=off  FilteringAndDerivatives=filter  SimscapeFilterOrder=2  InputFilterTimeConstant=0.001  UdotUserProvided=0
  Simulink-PS Converter2 : nesl_utility/Simulink-PS Converter  PhysicalDomain=network_engine_domain  SubClassName=ps_input  LeftPortType=input  RightPortType=output  PseudoPeriodic=off  Frequencies=[]  NoiseDistribution=none  NoiseParameters=[]  Unit=deg  AffineConversion=off  FilteringAndDerivatives=filter  SimscapeFilterOrder=2  InputFilterTimeConstant=0.001  UdotUserProvided=0
  Simulink-PS Converter3 : nesl_utility/Simulink-PS Converter  PhysicalDomain=network_engine_domain  SubClassName=ps_input  LeftPortType=input  RightPortType=output  PseudoPeriodic=off  Frequencies=[]  NoiseDistribution=none  NoiseParameters=[]  Unit=deg  AffineConversion=off  FilteringAndDerivatives=filter  SimscapeFilterOrder=2  InputFilterTimeConstant=0.001  UdotUserProvided=0
  Mafsal 1 : PMIOPort  Side=Right
  Mafsal 2 : PMIOPort  Port=2  Side=Right
  Mafsal 3 : PMIOPort  Port=3  Side=Right
  wires:
  MATLAB Function2/1(angles) -> Demux1/1
  Demux1/1 -> Gain/1
  Demux1/3 -> Simulink-PS Converter2/1
  Demux1/2 -> Simulink-PS Converter1/1
  MATLAB Function1/1(pos) -> MATLAB Function2/1(pos)
  Constant/1 -> MATLAB Function1/2(phase_offset)
  Clock1/1 -> MATLAB Function1/1(t)
  H_hedef/1 -> MATLAB Function1/3(H_hedef)
  Gain/1 -> Simulink-PS Converter3/1
  connections:
  Simulink-PS Converter2/RConn1 -- Mafsal 3/RConn1
  Simulink-PS Converter1/RConn1 -- Mafsal 2/RConn1
  Mafsal 1/RConn1 -- Simulink-PS Converter3/RConn1

== system Koudruped_simcape/Left Front Step1 ==
  H_hedef : Inport
  Clock1 : Clock
  Constant : Constant  Value=0.5
  Demux1 : Demux  Outputs=3
  Gain : Gain  Gain=-1
  MATLAB Function1 : MATLAB Function  TreatAsAtomicUnit=on
  MATLAB Function2 : MATLAB Function  TreatAsAtomicUnit=on
  Simulink-PS Converter1 : nesl_utility/Simulink-PS Converter  PhysicalDomain=network_engine_domain  SubClassName=ps_input  LeftPortType=input  RightPortType=output  PseudoPeriodic=off  Frequencies=[]  NoiseDistribution=none  NoiseParameters=[]  Unit=deg  AffineConversion=off  FilteringAndDerivatives=filter  SimscapeFilterOrder=2  InputFilterTimeConstant=0.001  UdotUserProvided=0
  Simulink-PS Converter2 : nesl_utility/Simulink-PS Converter  PhysicalDomain=network_engine_domain  SubClassName=ps_input  LeftPortType=input  RightPortType=output  PseudoPeriodic=off  Frequencies=[]  NoiseDistribution=none  NoiseParameters=[]  Unit=deg  AffineConversion=off  FilteringAndDerivatives=filter  SimscapeFilterOrder=2  InputFilterTimeConstant=0.001  UdotUserProvided=0
  Simulink-PS Converter3 : nesl_utility/Simulink-PS Converter  PhysicalDomain=network_engine_domain  SubClassName=ps_input  LeftPortType=input  RightPortType=output  PseudoPeriodic=off  Frequencies=[]  NoiseDistribution=none  NoiseParameters=[]  Unit=deg  AffineConversion=off  FilteringAndDerivatives=filter  SimscapeFilterOrder=2  InputFilterTimeConstant=0.001  UdotUserProvided=0
  Mafsal 1 : PMIOPort  Side=Right
  Mafsal 2 : PMIOPort  Port=2  Side=Right
  Mafsal 3 : PMIOPort  Port=3  Side=Right
  wires:
  MATLAB Function2/1(angles) -> Demux1/1
  Demux1/1 -> Gain/1
  Demux1/2 -> Simulink-PS Converter1/1
  MATLAB Function1/1(pos) -> MATLAB Function2/1(pos)
  Constant/1 -> MATLAB Function1/2(phase_offset)
  Clock1/1 -> MATLAB Function1/1(t)
  H_hedef/1 -> MATLAB Function1/3(H_hedef)
  Gain/1 -> Simulink-PS Converter3/1
  Demux1/3 -> Simulink-PS Converter2/1
  connections:
  Simulink-PS Converter2/RConn1 -- Mafsal 3/RConn1
  Simulink-PS Converter1/RConn1 -- Mafsal 2/RConn1
  Mafsal 1/RConn1 -- Simulink-PS Converter3/RConn1

== system Koudruped_simcape/Left Front Step2 ==
  H_hedef : Inport
  Clock1 : Clock
  Constant : Constant  Value=0.5
  Demux1 : Demux  Outputs=3
  Gain : Gain  Gain=-1
  MATLAB Function1 : MATLAB Function  TreatAsAtomicUnit=on
  MATLAB Function2 : MATLAB Function  TreatAsAtomicUnit=on
  Simulink-PS Converter1 : nesl_utility/Simulink-PS Converter  PhysicalDomain=network_engine_domain  SubClassName=ps_input  LeftPortType=input  RightPortType=output  PseudoPeriodic=off  Frequencies=[]  NoiseDistribution=none  NoiseParameters=[]  Unit=deg  AffineConversion=off  FilteringAndDerivatives=filter  SimscapeFilterOrder=2  InputFilterTimeConstant=0.001  UdotUserProvided=0
  Simulink-PS Converter2 : nesl_utility/Simulink-PS Converter  PhysicalDomain=network_engine_domain  SubClassName=ps_input  LeftPortType=input  RightPortType=output  PseudoPeriodic=off  Frequencies=[]  NoiseDistribution=none  NoiseParameters=[]  Unit=deg  AffineConversion=off  FilteringAndDerivatives=filter  SimscapeFilterOrder=2  InputFilterTimeConstant=0.001  UdotUserProvided=0
  Simulink-PS Converter3 : nesl_utility/Simulink-PS Converter  PhysicalDomain=network_engine_domain  SubClassName=ps_input  LeftPortType=input  RightPortType=output  PseudoPeriodic=off  Frequencies=[]  NoiseDistribution=none  NoiseParameters=[]  Unit=deg  AffineConversion=off  FilteringAndDerivatives=filter  SimscapeFilterOrder=2  InputFilterTimeConstant=0.001  UdotUserProvided=0
  Mafsal 1 : PMIOPort  Side=Right
  Mafsal 2 : PMIOPort  Port=2  Side=Right
  Mafsal 3 : PMIOPort  Port=3  Side=Right
  wires:
  MATLAB Function2/1(angles) -> Demux1/1
  Demux1/1 -> Gain/1
  Demux1/2 -> Simulink-PS Converter1/1
  MATLAB Function1/1(pos) -> MATLAB Function2/1(pos)
  Constant/1 -> MATLAB Function1/2(phase_offset)
  Clock1/1 -> MATLAB Function1/1(t)
  H_hedef/1 -> MATLAB Function1/3(H_hedef)
  Gain/1 -> Simulink-PS Converter3/1
  Demux1/3 -> Simulink-PS Converter2/1
  connections:
  Simulink-PS Converter2/RConn1 -- Mafsal 3/RConn1
  Simulink-PS Converter1/RConn1 -- Mafsal 2/RConn1
  Mafsal 1/RConn1 -- Simulink-PS Converter3/RConn1

== system Koudruped_simcape/Left Front Step3 ==
  H_hedef : Inport
  Clock1 : Clock
  Constant : Constant  Value=0.5
  Demux1 : Demux  Outputs=3
  Gain : Gain  Gain=-1
  MATLAB Function1 : MATLAB Function  TreatAsAtomicUnit=on
  MATLAB Function2 : MATLAB Function  TreatAsAtomicUnit=on
  Simulink-PS Converter1 : nesl_utility/Simulink-PS Converter  PhysicalDomain=network_engine_domain  SubClassName=ps_input  LeftPortType=input  RightPortType=output  PseudoPeriodic=off  Frequencies=[]  NoiseDistribution=none  NoiseParameters=[]  Unit=deg  AffineConversion=off  FilteringAndDerivatives=filter  SimscapeFilterOrder=2  InputFilterTimeConstant=0.001  UdotUserProvided=0
  Simulink-PS Converter2 : nesl_utility/Simulink-PS Converter  PhysicalDomain=network_engine_domain  SubClassName=ps_input  LeftPortType=input  RightPortType=output  PseudoPeriodic=off  Frequencies=[]  NoiseDistribution=none  NoiseParameters=[]  Unit=deg  AffineConversion=off  FilteringAndDerivatives=filter  SimscapeFilterOrder=2  InputFilterTimeConstant=0.001  UdotUserProvided=0
  Simulink-PS Converter3 : nesl_utility/Simulink-PS Converter  PhysicalDomain=network_engine_domain  SubClassName=ps_input  LeftPortType=input  RightPortType=output  PseudoPeriodic=off  Frequencies=[]  NoiseDistribution=none  NoiseParameters=[]  Unit=deg  AffineConversion=off  FilteringAndDerivatives=filter  SimscapeFilterOrder=2  InputFilterTimeConstant=0.001  UdotUserProvided=0
  Mafsal 1 : PMIOPort  Side=Right
  Mafsal 2 : PMIOPort  Port=2  Side=Right
  Mafsal 3 : PMIOPort  Port=3  Side=Right
  wires:
  MATLAB Function2/1(angles) -> Demux1/1
  Demux1/1 -> Gain/1
  Demux1/2 -> Simulink-PS Converter1/1
  MATLAB Function1/1(pos) -> MATLAB Function2/1(pos)
  Constant/1 -> MATLAB Function1/2(phase_offset)
  Clock1/1 -> MATLAB Function1/1(t)
  H_hedef/1 -> MATLAB Function1/3(H_hedef)
  Gain/1 -> Simulink-PS Converter3/1
  Demux1/3 -> Simulink-PS Converter2/1
  connections:
  Simulink-PS Converter2/RConn1 -- Mafsal 3/RConn1
  Simulink-PS Converter1/RConn1 -- Mafsal 2/RConn1
  Mafsal 1/RConn1 -- Simulink-PS Converter3/RConn1

== system Koudruped_simcape/Right Back Step ==
  H_hedef : Inport
  Clock1 : Clock
  Constant : Constant  Value=0.5
  Demux1 : Demux  Outputs=3
  MATLAB Function1 : MATLAB Function  TreatAsAtomicUnit=on
  MATLAB Function2 : MATLAB Function  TreatAsAtomicUnit=on
  Simulink-PS Converter1 : nesl_utility/Simulink-PS Converter  PhysicalDomain=network_engine_domain  SubClassName=ps_input  LeftPortType=input  RightPortType=output  PseudoPeriodic=off  Frequencies=[]  NoiseDistribution=none  NoiseParameters=[]  Unit=deg  AffineConversion=off  FilteringAndDerivatives=filter  SimscapeFilterOrder=2  InputFilterTimeConstant=0.001  UdotUserProvided=0
  Simulink-PS Converter2 : nesl_utility/Simulink-PS Converter  PhysicalDomain=network_engine_domain  SubClassName=ps_input  LeftPortType=input  RightPortType=output  PseudoPeriodic=off  Frequencies=[]  NoiseDistribution=none  NoiseParameters=[]  Unit=deg  AffineConversion=off  FilteringAndDerivatives=filter  SimscapeFilterOrder=2  InputFilterTimeConstant=0.001  UdotUserProvided=0
  Simulink-PS Converter3 : nesl_utility/Simulink-PS Converter  PhysicalDomain=network_engine_domain  SubClassName=ps_input  LeftPortType=input  RightPortType=output  PseudoPeriodic=off  Frequencies=[]  NoiseDistribution=none  NoiseParameters=[]  Unit=deg  AffineConversion=off  FilteringAndDerivatives=filter  SimscapeFilterOrder=2  InputFilterTimeConstant=0.001  UdotUserProvided=0
  Mafsal 1 : PMIOPort  Side=Right
  Mafsal 2 : PMIOPort  Port=2  Side=Right
  Mafsal 3 : PMIOPort  Port=3  Side=Right
  wires:
  Clock1/1 -> MATLAB Function1/1(t)
  Constant/1 -> MATLAB Function1/2(phase_offset)
  MATLAB Function1/1(pos) -> MATLAB Function2/1(pos)
  Demux1/2 -> Simulink-PS Converter1/1
  Demux1/3 -> Simulink-PS Converter2/1
  Demux1/1 -> Simulink-PS Converter3/1
  MATLAB Function2/1(angles) -> Demux1/1
  H_hedef/1 -> MATLAB Function1/3(H_hedef)
  connections:
  Mafsal 1/RConn1 -- Simulink-PS Converter3/RConn1
  Simulink-PS Converter1/RConn1 -- Mafsal 2/RConn1
  Simulink-PS Converter2/RConn1 -- Mafsal 3/RConn1

== system Koudruped_simcape/Right Back Step1 ==
  H_hedef : Inport
  Clock1 : Clock
  Constant : Constant  Value=0.5
  Demux1 : Demux  Outputs=3
  MATLAB Function1 : MATLAB Function  TreatAsAtomicUnit=on
  MATLAB Function2 : MATLAB Function  TreatAsAtomicUnit=on
  Simulink-PS Converter1 : nesl_utility/Simulink-PS Converter  PhysicalDomain=network_engine_domain  SubClassName=ps_input  LeftPortType=input  RightPortType=output  PseudoPeriodic=off  Frequencies=[]  NoiseDistribution=none  NoiseParameters=[]  Unit=deg  AffineConversion=off  FilteringAndDerivatives=filter  SimscapeFilterOrder=2  InputFilterTimeConstant=0.001  UdotUserProvided=0
  Simulink-PS Converter2 : nesl_utility/Simulink-PS Converter  PhysicalDomain=network_engine_domain  SubClassName=ps_input  LeftPortType=input  RightPortType=output  PseudoPeriodic=off  Frequencies=[]  NoiseDistribution=none  NoiseParameters=[]  Unit=deg  AffineConversion=off  FilteringAndDerivatives=filter  SimscapeFilterOrder=2  InputFilterTimeConstant=0.001  UdotUserProvided=0
  Simulink-PS Converter3 : nesl_utility/Simulink-PS Converter  PhysicalDomain=network_engine_domain  SubClassName=ps_input  LeftPortType=input  RightPortType=output  PseudoPeriodic=off  Frequencies=[]  NoiseDistribution=none  NoiseParameters=[]  Unit=deg  AffineConversion=off  FilteringAndDerivatives=filter  SimscapeFilterOrder=2  InputFilterTimeConstant=0.001  UdotUserProvided=0
  Mafsal 1 : PMIOPort  Side=Right
  Mafsal 2 : PMIOPort  Port=2  Side=Right
  Mafsal 3 : PMIOPort  Port=3  Side=Right
  wires:
  Clock1/1 -> MATLAB Function1/1(t)
  Constant/1 -> MATLAB Function1/2(phase_offset)
  MATLAB Function1/1(pos) -> MATLAB Function2/1(pos)
  Demux1/2 -> Simulink-PS Converter1/1
  Demux1/1 -> Simulink-PS Converter3/1
  MATLAB Function2/1(angles) -> Demux1/1
  H_hedef/1 -> MATLAB Function1/3(H_hedef)
  Demux1/3 -> Simulink-PS Converter2/1
  connections:
  Mafsal 1/RConn1 -- Simulink-PS Converter3/RConn1
  Simulink-PS Converter1/RConn1 -- Mafsal 2/RConn1
  Simulink-PS Converter2/RConn1 -- Mafsal 3/RConn1

== system Koudruped_simcape/Right Back Step2 ==
  H_hedef : Inport
  Clock1 : Clock
  Constant : Constant  Value=0.5
  Demux1 : Demux  Outputs=3
  Display : Display
  MATLAB Function1 : MATLAB Function  TreatAsAtomicUnit=on
  MATLAB Function2 : MATLAB Function  TreatAsAtomicUnit=on
  Right Back : Scope
      settings: ActiveDisplayYMinimum=-1  ActiveDisplayYMaximum=1  DataLoggingVariableName=ScopeData3
  Right Back1 : Scope
      settings: ActiveDisplayYMinimum=-1  ActiveDisplayYMaximum=1  DataLoggingVariableName=ScopeData6
  Simulink-PS Converter1 : nesl_utility/Simulink-PS Converter  PhysicalDomain=network_engine_domain  SubClassName=ps_input  LeftPortType=input  RightPortType=output  PseudoPeriodic=off  Frequencies=[]  NoiseDistribution=none  NoiseParameters=[]  Unit=deg  AffineConversion=off  FilteringAndDerivatives=filter  SimscapeFilterOrder=2  InputFilterTimeConstant=0.001  UdotUserProvided=0
  Simulink-PS Converter2 : nesl_utility/Simulink-PS Converter  PhysicalDomain=network_engine_domain  SubClassName=ps_input  LeftPortType=input  RightPortType=output  PseudoPeriodic=off  Frequencies=[]  NoiseDistribution=none  NoiseParameters=[]  Unit=deg  AffineConversion=off  FilteringAndDerivatives=filter  SimscapeFilterOrder=2  InputFilterTimeConstant=0.001  UdotUserProvided=0
  Simulink-PS Converter3 : nesl_utility/Simulink-PS Converter  PhysicalDomain=network_engine_domain  SubClassName=ps_input  LeftPortType=input  RightPortType=output  PseudoPeriodic=off  Frequencies=[]  NoiseDistribution=none  NoiseParameters=[]  Unit=deg  AffineConversion=off  FilteringAndDerivatives=filter  SimscapeFilterOrder=2  InputFilterTimeConstant=0.001  UdotUserProvided=0
  Mafsal 1 : PMIOPort  Side=Right
  Mafsal 2 : PMIOPort  Port=2  Side=Right
  Mafsal 3 : PMIOPort  Port=3  Side=Right
  wires:
  Clock1/1 -> MATLAB Function1/1(t)
  Constant/1 -> MATLAB Function1/2(phase_offset)
  MATLAB Function1/1(pos) -> MATLAB Function2/1(pos)
  Demux1/2 -> Simulink-PS Converter1/1
  Demux1/1 -> Simulink-PS Converter3/1
  MATLAB Function2/1(angles) -> Demux1/1
  H_hedef/1 -> Display/1, Right Back/1, MATLAB Function1/3(H_hedef)
  Demux1/3 -> Right Back1/1, Simulink-PS Converter2/1
  connections:
  Mafsal 1/RConn1 -- Simulink-PS Converter3/RConn1
  Simulink-PS Converter1/RConn1 -- Mafsal 2/RConn1
  Simulink-PS Converter2/RConn1 -- Mafsal 3/RConn1

== system Koudruped_simcape/Right Back Step3 ==
  H_hedef : Inport
  Clock1 : Clock
  Constant : Constant  Value=0.5
  Demux1 : Demux  Outputs=3
  MATLAB Function1 : MATLAB Function  TreatAsAtomicUnit=on
  MATLAB Function2 : MATLAB Function  TreatAsAtomicUnit=on
  Simulink-PS Converter1 : nesl_utility/Simulink-PS Converter  PhysicalDomain=network_engine_domain  SubClassName=ps_input  LeftPortType=input  RightPortType=output  PseudoPeriodic=off  Frequencies=[]  NoiseDistribution=none  NoiseParameters=[]  Unit=deg  AffineConversion=off  FilteringAndDerivatives=filter  SimscapeFilterOrder=2  InputFilterTimeConstant=0.001  UdotUserProvided=0
  Simulink-PS Converter2 : nesl_utility/Simulink-PS Converter  PhysicalDomain=network_engine_domain  SubClassName=ps_input  LeftPortType=input  RightPortType=output  PseudoPeriodic=off  Frequencies=[]  NoiseDistribution=none  NoiseParameters=[]  Unit=deg  AffineConversion=off  FilteringAndDerivatives=filter  SimscapeFilterOrder=2  InputFilterTimeConstant=0.001  UdotUserProvided=0
  Simulink-PS Converter3 : nesl_utility/Simulink-PS Converter  PhysicalDomain=network_engine_domain  SubClassName=ps_input  LeftPortType=input  RightPortType=output  PseudoPeriodic=off  Frequencies=[]  NoiseDistribution=none  NoiseParameters=[]  Unit=deg  AffineConversion=off  FilteringAndDerivatives=filter  SimscapeFilterOrder=2  InputFilterTimeConstant=0.001  UdotUserProvided=0
  Mafsal 1 : PMIOPort  Side=Right
  Mafsal 2 : PMIOPort  Port=2  Side=Right
  Mafsal 3 : PMIOPort  Port=3  Side=Right
  wires:
  Clock1/1 -> MATLAB Function1/1(t)
  Constant/1 -> MATLAB Function1/2(phase_offset)
  MATLAB Function1/1(pos) -> MATLAB Function2/1(pos)
  Demux1/2 -> Simulink-PS Converter1/1
  Demux1/1 -> Simulink-PS Converter3/1
  MATLAB Function2/1(angles) -> Demux1/1
  H_hedef/1 -> MATLAB Function1/3(H_hedef)
  Demux1/3 -> Simulink-PS Converter2/1
  connections:
  Mafsal 1/RConn1 -- Simulink-PS Converter3/RConn1
  Simulink-PS Converter1/RConn1 -- Mafsal 2/RConn1
  Simulink-PS Converter2/RConn1 -- Mafsal 3/RConn1
